simulink model "YMBOX_Control_Core"  (R2024b)
settings: Solver=FixedStepDiscrete  StartTime=0.0  StopTime=3  RelTol=1e-3
PreLoadFcn:
  | run(fullfile(fileparts(get_param(bdroot,'FileName')), 'YMBOX_Deluxe_init.m'));
InitFcn:
  | YMBOX_InitializeModel('core',bdroot);
model workspace (MAT data in the model file):
  KuMDAS_ObserverBuildVariant : Simulink.Parameter (value not decoded)
undefined symbols (not defined in the file or in its folder): CeMDSM_DrvModeIfStart_enum, CeMDSM_DrvModeSpdSens_enum, CeMDSM_DrvModeSpdSmo_enum, CeMDSM_DrvModeTrq_enum, Cf_CONTROL_TASK_TIME_S, KbMDAS_SmoDeadTimeCompEnable_flg, KbMDSA_ActiveInverterCompEnable_flg, KbMDSA_UnifiedVoltageLimitEnable_flg, KbMDSP_DCBusVoltReportFilterEnable_flg, KbMDTM_DAxisPriorityInFW_flg, KbMDTM_FieldWeakeningEnable_flg, KbMDTM_FinalIqAntiWindupEnable_flg, KbMDTM_SensorlessFieldWeakeningEnable_flg, KbMDTM_TorquePriorityBelowBase_flg, KbMDTM_UnifiedConstraintEnable_flg, KfMDAS_ControlCountToElecRad_NULL, KfMDAS_IfAccel_rpms, KfMDAS_IfAlignTime_s, KfMDAS_IfBlendTime_s, KfMDAS_IfSwitchSpd_rpm, KfMDAS_NativeCountToMechRad_NULL, KfMDAS_ObserverExitRatio_NULL, KfMDAS_SlsCtrlPeriod_s, KfMDAS_SlsEAngleInit_rad, KfMDAS_SlsElecSpdMax_rads, KfMDAS_SlsElecSpdMin_rads, KfMDAS_SlsTwoPi_rad, KfMDAS_SmoAngleOffset_rad, KfMDAS_SmoCurrentZohCoefA_NULL, KfMDAS_SmoCurrentZohCoefB_AperV, KfMDAS_SmoDeadTimeCurrentBoundary_A, KfMDAS_SmoDeadTimeDuty_NULL, KfMDAS_SmoDeadTimePolarity_NULL, KfMDAS_SmoDeviceDrop_V, KfMDAS_SmoEmfLpfCoefA_NULL, KfMDAS_SmoEmfLpfCoefB_NULL, KfMDAS_SmoEmfLpfInvPole_s, KfMDAS_SmoErrBoundaryMax_A, KfMDAS_SmoErrBoundarySpan_A, KfMDAS_SmoGainSchedAlpha_NULL, KfMDAS_SmoGainSchedAngleComp_rad, KfMDAS_SmoGainSchedEmfLow_V, KfMDAS_SmoGainSchedInvSpan_PerV, KfMDAS_SmoLdMinusLq_H, KfMDAS_SmoPllKiTs_NULL, KfMDAS_SmoPllKp_NULL, KfMDAS_SmoPllMinEmf_V, KfMDAS_SmoPllSpeedLpfAlpha_NULL, KfMDAS_SmoSlideGainMin_V, KfMDAS_SmoSlideGainSpan_V, KfMDAS_SmoSwitchSpd_rpm, KfMDAS_SmoTotalDelay_s, KfMDCC_DqSoftwareOverCurrentThreshold_A, KfMDCC_PiKcTsId_NULL, KfMDCC_PiKcTsIq_NULL, KfMDCC_PiKiTsId_NULL, KfMDCC_PiKiTsIq_NULL, KfMDCC_PiKpValueId_NULL, KfMDCC_PiKpValueIq_NULL, KfMDCC_PwmFreq_Hz ... (+84)
libraries: YMBOX_SharedMath_Lib x11, spsabctoAlphaBetaZeroLib x1
(part 8 of 8)

== matlab function YMBOX_Control_Core/MDFM/FaultState ==
  data: hwFaultActive input; stopRequest output; hwFaultCode input; platformFaultMask input; platformWarningMask input; platformTorqueLimit input; phaseUErr input; phaseVErr input; phaseWErr input; phaseSoftwareOverCurrent input; dqSoftwareOverCurrent input; dcOverVoltage input; dcUnderVoltage input; commandTimeout input; clearFaultRequest input; historyReadIndex input; mcuEnable input; vdc input; iu input; iv input; iw input; modeReq input; spdCmd input; trqCmd input; clearHoldCount input; faultLatched output; activeFaultCode output; rawFaultMask output; latchedFaultMask output; lastHwFaultCode output; faultOccurrence output; snapshotVdc output; snapshotIu output; snapshotIv output; snapshotIw output; snapshotModeReq output; snapshotSpdCmd output; snapshotTrqCmd output; clearReady output; pwmDisableRequest output; piResetRequest output; torqueLimitFactor output; warningActive output; faultAction output; firstFaultCode output; platformFaultMaskOut output; platformWarningMaskOut output; clearRequestRequired output; clearRejected output; historyCount output; historyWriteIndex output; historyReadValid output; historyReadCode output; historyReadAction output; historyReadMask output; historyReadPlatformMask output; historyReadVdc output; historyReadMaxCurrent output; historyReadMode output; historyReadSpdCmd output; historyReadTrqCmd output
function [stopRequest, faultLatched, activeFaultCode, rawFaultMask, latchedFaultMask, lastHwFaultCode, faultOccurrence, snapshotVdc, snapshotIu, snapshotIv, snapshotIw, snapshotModeReq, snapshotSpdCmd, snapshotTrqCmd, clearReady, pwmDisableRequest, piResetRequest, torqueLimitFactor, warningActive, faultAction, firstFaultCode, platformFaultMaskOut, platformWarningMaskOut, clearRequestRequired, clearRejected, historyCount, historyWriteIndex, historyReadValid, historyReadCode, historyReadAction, historyReadMask, historyReadPlatformMask, historyReadVdc, historyReadMaxCurrent, historyReadMode, historyReadSpdCmd, historyReadTrqCmd] = MDFM_Fault_State_Manager(hwFaultActive, hwFaultCode, platformFaultMask, platformWarningMask, platformTorqueLimit, phaseUErr, phaseVErr, phaseWErr, phaseSoftwareOverCurrent, dqSoftwareOverCurrent, dcOverVoltage, dcUnderVoltage, commandTimeout, clearFaultRequest, historyReadIndex, mcuEnable, vdc, iu, iv, iw, modeReq, spdCmd, trqCmd, clearHoldCount)
%#codegen
% Application-level fault arbitration, recovery, and event history.
% Hardware-specific asynchronous shutdown remains in the platform HAL.

persistent latchedState firstCodePersist latchedMaskPersist
persistent hwCodePersist occurrencePersist clearCountPersist clearRequestPersist
persistent snapVdcPersist snapIuPersist snapIvPersist snapIwPersist
persistent snapModePersist snapSpdPersist snapTrqPersist
persistent previousTripMask previousLocalWarningMask previousPlatformFaultMask previousPlatformWarningMask
persistent historyCountPersist historyWritePersist
persistent historyCodePersist historyActionPersist historyMaskPersist
persistent historyPlatformMaskPersist historyVdcPersist historyMaxCurrentPersist
persistent historyModePersist historySpdPersist historyTrqPersist

if isempty(latchedState)
    latchedState = false;
    firstCodePersist = uint16(0);
    latchedMaskPersist = uint32(0);
    hwCodePersist = uint16(0);
    occurrencePersist = uint32(0);
    clearCountPersist = uint32(0);
    clearRequestPersist = false;
    snapVdcPersist = single(0);
    snapIuPersist = single(0);
    snapIvPersist = single(0);
    snapIwPersist = single(0);
    snapModePersist = uint16(0);
    snapSpdPersist = single(0);
    snapTrqPersist = single(0);
    previousTripMask = uint32(0);
    previousLocalWarningMask = uint32(0);
    previousPlatformFaultMask = uint32(0);
    previousPlatformWarningMask = uint32(0);
    historyCountPersist = uint8(0);
    historyWritePersist = uint8(0);
    historyCodePersist = zeros(1, 8, 'uint16');
    historyActionPersist = zeros(1, 8, 'uint8');
    historyMaskPersist = zeros(1, 8, 'uint32');
    historyPlatformMaskPersist = zeros(1, 8, 'uint32');
    historyVdcPersist = zeros(1, 8, 'single');
    historyMaxCurrentPersist = zeros(1, 8, 'single');
    historyModePersist = zeros(1, 8, 'uint16');
    historySpdPersist = zeros(1, 8, 'single');
    historyTrqPersist = zeros(1, 8, 'single');
end

dqSoftwareOverCurrentBit = bitshift(uint32(1), 10);
tripMaskConstant = bitor(uint32(399), dqSoftwareOverCurrentBit);
phaseMaskConstant = uint32(112);
manualClearMask = bitor(uint32(243), dqSoftwareOverCurrentBit);
warningBit = bitshift(uint32(1), 9);
rawFaultMask = uint32(0);

if hwFaultActive
    rawFaultMask = bitor(rawFaultMask, bitshift(uint32(1), 0));
    hwCodePersist = uint16(hwFaultCode);
end
if dcOverVoltage
    rawFaultMask = bitor(rawFaultMask, bitshift(uint32(1), 2));
end
if phaseUErr
    rawFaultMask = bitor(rawFaultMask, bitshift(uint32(1), 4));
end
if phaseVErr
    rawFaultMask = bitor(rawFaultMask, bitshift(uint32(1), 5));
end
if phaseWErr
    rawFaultMask = bitor(rawFaultMask, bitshift(uint32(1), 6));
end
phaseErrorMask = bitand(rawFaultMask, phaseMaskConstant);
phaseErrorCount = uint8(phaseUErr) + uint8(phaseVErr) + uint8(phaseWErr);
singlePhaseWarning = (phaseErrorCount == uint8(1));
multiplePhaseFault = (phaseErrorCount >= uint8(2));
if platformFaultMask ~= uint32(0)
    rawFaultMask = bitor(rawFaultMask, bitshift(uint32(1), 7));
end
if mcuEnable
    if phaseSoftwareOverCurrent
        rawFaultMask = bitor(rawFaultMask, bitshift(uint32(1), 1));
    end
    if dqSoftwareOverCurrent
        rawFaultMask = bitor(rawFaultMask, dqSoftwareOverCurrentBit);
    end
    if dcUnderVoltage
        rawFaultMask = bitor(rawFaultMask, bitshift(uint32(1), 3));
    end
    if commandTimeout
        rawFaultMask = bitor(rawFaultMask, bitshift(uint32(1), 8));
    end
end

limitedTorqueFactor = min(max(single(platformTorqueLimit), single(0)), single(1));
warningActive = (platformWarningMask ~= uint32(0)) || ...
    (limitedTorqueFactor < single(1)) || singlePhaseWarning;
if warningActive
    rawFaultMask = bitor(rawFaultMask, warningBit);
end

rawTripMask = bitand(rawFaultMask, tripMaskConstant);
if multiplePhaseFault
    rawTripMask = bitor(rawTripMask, phaseErrorMask);
end
localWarningMask = uint32(0);
if singlePhaseWarning
    localWarningMask = bitor(phaseErrorMask, warningBit);
end
newTripBits = bitand(rawTripMask, bitcmp(previousTripMask));
newLocalWarningBits = bitand(localWarningMask, bitcmp(previousLocalWarningMask));
newPlatformFaultBits = bitand(uint32(platformFaultMask), bitcmp(previousPlatformFaultMask));
newPlatformWarningBits = bitand(uint32(platformWarningMask), bitcmp(previousPlatformWarningMask));
newManualBits = bitand(newTripBits, manualClearMask);

if newManualBits ~= uint32(0)
    clearRequestPersist = false;
end

if (~latchedState) && (rawTripMask ~= uint32(0))
    latchedState = true;
    latchedMaskPersist = rawTripMask;
    firstCodePersist = localSelectFaultCode(rawTripMask);
    clearCountPersist = uint32(0);
    snapVdcPersist = single(vdc);
    snapIuPersist = single(iu);
    snapIvPersist = single(iv);
    snapIwPersist = single(iw);
    snapModePersist = uint16(modeReq);
    snapSpdPersist = single(spdCmd);
    snapTrqPersist = single(trqCmd);
elseif latchedState
    latchedMaskPersist = bitor(latchedMaskPersist, rawTripMask);
end

clearRequestRequired = latchedState && ...
    (bitand(latchedMaskPersist, manualClearMask) ~= uint32(0));
clearCondition = latchedState && (~mcuEnable) && ...
    (rawTripMask == uint32(0));

clearRejected = clearFaultRequest && (~clearCondition);
if clearFaultRequest && clearCondition
    clearRequestPersist = true;
end
clearPermission = (~clearRequestRequired) || clearRequestPersist;
clearReady = clearCondition && clearPermission;

if clearReady
    if clearCountPersist < uint32(clearHoldCount)
        clearCountPersist = clearCountPersist + uint32(1);
    end
    if clearCountPersist >= uint32(clearHoldCount)
        latchedState = false;
        firstCodePersist = uint16(0);
        latchedMaskPersist = uint32(0);
        clearCountPersist = uint32(0);
        clearRequestPersist = false;
    end
else
    clearCountPersist = uint32(0);
end

historyEvent = (newTripBits ~= uint32(0)) || ...
    (newLocalWarningBits ~= uint32(0)) || ...
    (newPlatformFaultBits ~= uint32(0)) || ...
    (newPlatformWarningBits ~= uint32(0));
if historyEvent
    eventMask = newTripBits;
    eventPlatformMask = bitor(newPlatformFaultBits, newPlatformWarningBits);
    if eventMask ~= uint32(0)
        eventCode = localSelectFaultCode(eventMask);
        eventAction = localSelectFaultAction(eventMask);
    elseif newLocalWarningBits ~= uint32(0)
        eventMask = newLocalWarningBits;
        eventCode = localSelectFaultCode(eventMask);
        eventAction = uint8(2);
    elseif newPlatformFaultBits ~= uint32(0)
        eventMask = bitshift(uint32(1), 7);
        eventCode = uint16(8);
        eventAction = uint8(4);
    else
        eventMask = warningBit;
        eventCode = uint16(10);
        eventAction = uint8(2);
    end

    historyIndex = uint8(historyWritePersist + uint8(1));
    historyCodePersist(historyIndex) = eventCode;
    historyActionPersist(historyIndex) = eventAction;
    historyMaskPersist(historyIndex) = eventMask;
    historyPlatformMaskPersist(historyIndex) = eventPlatformMask;
    historyVdcPersist(historyIndex) = single(vdc);
    historyMaxCurrentPersist(historyIndex) = max(abs(single(iu)), ...
        max(abs(single(iv)), abs(single(iw))));
    historyModePersist(historyIndex) = uint16(modeReq);
    historySpdPersist(historyIndex) = single(spdCmd);
    historyTrqPersist(historyIndex) = single(trqCmd);

    if historyWritePersist >= uint8(7)
        historyWritePersist = uint8(0);
    else
        historyWritePersist = historyWritePersist + uint8(1);
    end
    if historyCountPersist < uint8(8)
        historyCountPersist = historyCountPersist + uint8(1);
    end
    if occurrencePersist < intmax('uint32')
        occurrencePersist = occurrencePersist + uint32(1);
    end
end

previousTripMask = rawTripMask;
previousLocalWarningMask = localWarningMask;
previousPlatformFaultMask = uint32(platformFaultMask);
previousPlatformWarningMask = uint32(platformWarningMask);

stopRequest = latchedState;
faultLatched = latchedState;
pwmDisableRequest = latchedState;
piResetRequest = latchedState;
latchedFaultMask = latchedMaskPersist;
firstFaultCode = firstCodePersist;
if latchedState
    activeFaultCode = localSelectFaultCode(latchedMaskPersist);
    faultAction = localSelectFaultAction(latchedMaskPersist);
    torqueLimitFactor = single(0);
elseif warningActive
    activeFaultCode = localSelectFaultCode(rawFaultMask);
    faultAction = uint8(2);
    torqueLimitFactor = limitedTorqueFactor;
else
    activeFaultCode = uint16(0);
    faultAction = uint8(0);
    torqueLimitFactor = single(1);
end

lastHwFaultCode = hwCodePersist;
faultOccurrence = occurrencePersist;
snapshotVdc = snapVdcPersist;
snapshotIu = snapIuPersist;
snapshotIv = snapIvPersist;
snapshotIw = snapIwPersist;
snapshotModeReq = snapModePersist;
snapshotSpdCmd = snapSpdPersist;
snapshotTrqCmd = snapTrqPersist;
platformFaultMaskOut = uint32(platformFaultMask);
platformWarningMaskOut = uint32(platformWarningMask);
historyCount = historyCountPersist;
historyWriteIndex = historyWritePersist;

historyReadValid = false;
historyReadCode = uint16(0);
historyReadAction = uint8(0);
historyReadMask = uint32(0);
historyReadPlatformMask = uint32(0);
historyReadVdc = single(0);
historyReadMaxCurrent = single(0);
historyReadMode = uint16(0);
historyReadSpdCmd = single(0);
historyReadTrqCmd = single(0);
if (historyReadIndex < historyCountPersist) && (historyReadIndex < uint8(8))
    physicalIndex = int16(historyWritePersist) - int16(1) - ...
        int16(historyReadIndex);
    while physicalIndex < int16(0)
        physicalIndex = physicalIndex + int16(8);
    end
    readIndex = uint8(physicalIndex + int16(1));
    historyReadValid = true;
    historyReadCode = historyCodePersist(readIndex);
    historyReadAction = historyActionPersist(readIndex);
    historyReadMask = historyMaskPersist(readIndex);
    historyReadPlatformMask = historyPlatformMaskPersist(readIndex);
    historyReadVdc = historyVdcPersist(readIndex);
    historyReadMaxCurrent = historyMaxCurrentPersist(readIndex);
    historyReadMode = historyModePersist(readIndex);
    historyReadSpdCmd = historySpdPersist(readIndex);
    historyReadTrqCmd = historyTrqPersist(readIndex);
end
end

function code = localSelectFaultCode(mask)
code = uint16(0);
if bitand(mask, bitshift(uint32(1), 0)) ~= uint32(0)
    code = uint16(1);
elseif bitand(mask, bitshift(uint32(1), 1)) ~= uint32(0)
    code = uint16(2);
elseif bitand(mask, bitshift(uint32(1), 10)) ~= uint32(0)
    code = uint16(11);
elseif bitand(mask, bitshift(uint32(1), 7)) ~= uint32(0)
    code = uint16(8);
elseif bitand(mask, bitshift(uint32(1), 4)) ~= uint32(0)
    code = uint16(5);
elseif bitand(mask, bitshift(uint32(1), 5)) ~= uint32(0)
    code = uint16(6);
elseif bitand(mask, bitshift(uint32(1), 6)) ~= uint32(0)
    code = uint16(7);
elseif bitand(mask, bitshift(uint32(1), 2)) ~= uint32(0)
    code = uint16(3);
elseif bitand(mask, bitshift(uint32(1), 3)) ~= uint32(0)
    code = uint16(4);
elseif bitand(mask, bitshift(uint32(1), 8)) ~= uint32(0)
    code = uint16(9);
elseif bitand(mask, bitshift(uint32(1), 9)) ~= uint32(0)
    code = uint16(10);
end
end

function action = localSelectFaultAction(mask)
immediateStopMask = bitor(uint32(131), bitshift(uint32(1), 10));
controlledStopMask = uint32(268);
phaseMask = bitand(mask, uint32(112));
warningMask = bitshift(uint32(1), 9);
phaseCount = uint8(0);
if bitand(phaseMask, bitshift(uint32(1), 4)) ~= uint32(0)
    phaseCount = phaseCount + uint8(1);
end
if bitand(phaseMask, bitshift(uint32(1), 5)) ~= uint32(0)
    phaseCount = phaseCount + uint8(1);
end
if bitand(phaseMask, bitshift(uint32(1), 6)) ~= uint32(0)
    phaseCount = phaseCount + uint8(1);
end
if bitand(mask, immediateStopMask) ~= uint32(0)
    action = uint8(4);
elseif phaseCount >= uint8(2)
    action = uint8(4);
elseif bitand(mask, controlledStopMask) ~= uint32(0)
    action = uint8(3);
elseif (phaseCount == uint8(1)) || ...
        (bitand(mask, warningMask) ~= uint32(0))
    action = uint8(2);
else
    action = uint8(0);
end
end

== matlab function YMBOX_Control_Core/MDTM/MDTM/MDTM_SMO/Switch Case Action Subsystem/SMO_SpeedPI_IqSeed ==
  data: modeCmd input; iqSeed output; modeReq input; angleDelta input; ifIq input; targetSpdRpm input; accelIqSeed input; adaptiveIqSeed input; pTerm input; blendWeight input; externalReset input; piTrackReset output
function [iqSeed,piTrackReset] = SMO_SpeedPI_IqSeed(modeCmd,modeReq,angleDelta,ifIq,targetSpdRpm,accelIqSeed,adaptiveIqSeed,pTerm,blendWeight,externalReset)
%#codegen
% Back-calculate the speed-PI integrator on every handover sample:
%     Iint = Iq_required - Kp*speed_error
% adaptiveIqSeed and blendWeight are bounded once at the MDTM boundary.
routeActive=(uint16(modeReq)==uint16(6)) && (uint16(modeCmd)==uint16(17));
if routeActive
    targetIq=adaptiveIqSeed;
    direction=single(0);
    if targetSpdRpm>=single(1e-3)
        direction=single(1);
    elseif targetSpdRpm<=single(-1e-3)
        direction=single(-1);
    end
    minimum=abs(accelIqSeed);
    if direction~=0.0 && direction*targetIq<minimum
        targetIq=direction*minimum;
    end
else
    targetIq=ifIq;
end
iqSeed=single(targetIq-pTerm);
blend=blendWeight;
% Pre-track the SMO speed PI throughout I/F and the whole blend.
handoverTracking=(routeActive || uint16(modeCmd)==uint16(16)) && ...
    blend<single(0.999);
piTrackReset=(externalReset~=0) || handoverTracking;
% angleDelta remains only for compatibility with the published interface.
end

== stateflow chart YMBOX_Control_Core/MDSM/MDSM_ModeManager/MDSM_RouteConfig_Variant/Route_Variant1_SMO/MDSM_ProductRouteConfig ==
  state RouteProductSMO
    en:
    [VbMDSM_RouteSupported_flg, VeMDSM_Stage1Mode_enum, ...
    VbMDSM_Stage1Ready_flg, VfMDSM_Stage1SwitchSpd_rpm, ...
    VuMDSM_Stage1Acquire_cnt, VbMDSM_Stage2Enable_flg, ...
    VeMDSM_Stage2Mode_enum, VbMDSM_Stage2Ready_flg, ...
    VfMDSM_Stage2SwitchSpd_rpm, VbMDSM_Stage2Fallback_flg] = ...
    YMBOX_SmoProductRouteConfig(VeMDSM_DrvModeReq_enum, ...
    VbMDAS_SmoReady_flg, KfMDAS_IfSwitchSpd_rpm, ...
    KfMDAS_SmoSwitchSpd_rpm, KuMDSM_ObserverLossConfirmCnt, ...
    KuMDSM_DirectHandoverCnt);
    du:
    [VbMDSM_RouteSupported_flg, VeMDSM_Stage1Mode_enum, ...
    VbMDSM_Stage1Ready_flg, VfMDSM_Stage1SwitchSpd_rpm, ...
    VuMDSM_Stage1Acquire_cnt, VbMDSM_Stage2Enable_flg, ...
    VeMDSM_Stage2Mode_enum, VbMDSM_Stage2Ready_flg, ...
    VfMDSM_Stage2SwitchSpd_rpm, VbMDSM_Stage2Fallback_flg] = ...
    YMBOX_SmoProductRouteConfig(VeMDSM_DrvModeReq_enum, ...
    VbMDAS_SmoReady_flg, KfMDAS_IfSwitchSpd_rpm, ...
    KfMDAS_SmoSwitchSpd_rpm, KuMDSM_ObserverLossConfirmCnt, ...
    KuMDSM_DirectHandoverCnt);
  (default) -> RouteProductSMO
  data: VeMDSM_DrvModeReq_enum input uint16; VbMDAS_SmoReady_flg input uint8; VbMDSM_RouteSupported_flg output boolean; VeMDSM_Stage1Mode_enum output uint16; VbMDSM_Stage1Ready_flg output boolean; VfMDSM_Stage1SwitchSpd_rpm output single; VuMDSM_Stage1Acquire_cnt output uint32; VbMDSM_Stage2Enable_flg output boolean; VeMDSM_Stage2Mode_enum output uint16; VbMDSM_Stage2Ready_flg output boolean; VfMDSM_Stage2SwitchSpd_rpm output single; VbMDSM_Stage2Fallback_flg output boolean; KfMDAS_IfSwitchSpd_rpm parameter single; KfMDAS_SmoSwitchSpd_rpm parameter single; KuMDSM_ObserverLossConfirmCnt parameter uint32; KuMDSM_DirectHandoverCnt parameter uint32
